simulink model "LabC_CompensatorOverRobot"  (R2017a)
settings: Solver=FixedStepDiscrete  StartTime=0.0  StopTime=inf  FixedStep=fSamplingPeriod  RelTol=1e-3  EnableMultiTasking=on
values from neighbouring files (symbols this model uses):
  Ad = [ ... (first row only)    [LabB_ObserverOverSimulator_Discrete_Parameters.m]
  Bd = [0,           0 ... (first row only)    [LabA_equations.m]    (also in LabB_ObserverOverSimulator_Discrete_Parameters.m = [)
  Cd = [ ... (first row only)    [LabB_ObserverOverSimulator_Discrete_Parameters.m]
  fGyroBias = 125.292978208    [GyroBias.mat]    (also in LabB_TuneTheGyro_SaveParameters.m = mean(afGyroBias.signals.values))
  fGyroConversionFactor = -1/131    (= -0.00763358778626)    [LabB_PIDOverRobot_Parameters.m]    (also in LoadRobotParameters.m = 0.00762939453125)
  fSamplingPeriod = 0.01    [LabB_CheckCommunications_Parameters.m]    (also in LabB_ControllerOverSimulator_Discrete_Parameters.m = 0.005; LabB_ObserverOverSimulator_Discrete_Parameters.m = 0.005; LabB_PIDOverRobot_Parameters.m = 0.005; LabB_TuneTheGyro_SaveParameters.m)
  fWheelRadius = 0.0216    [LabB_PIDOverRobot_Parameters.m]    (also in LoadRobotParameters.m)
  iNumberOfEncoderSteps = 720    [LabB_PIDOverRobot_Parameters.m]    (also in LoadRobotParameters.m)
  Kd = [-8.1792  -49.1223  -71.4928  -11.5909]    [LabB_ControllerOverSimulator_Discrete_Parameters.m]
  Ld = [ ... (first row only)    [LabB_ObserverOverSimulator_Discrete_Parameters.m]
  Md1 = [ ... (first row only)    [LabB_ObserverOverSimulator_Discrete_Parameters.m]
  Md2 = [ ... (first row only)    [LabB_ObserverOverSimulator_Discrete_Parameters.m]
  Md3 = 1.0e+03 * [ ... (first row only)    [LabB_ObserverOverSimulator_Discrete_Parameters.m]
  Md4 = [ ... (first row only)    [LabB_ObserverOverSimulator_Discrete_Parameters.m]
  Md5 = 1.0e+03 * [ ... (first row only)    [LabB_ObserverOverSimulator_Discrete_Parameters.m]
  Md6 = [ ... (first row only)    [LabB_ObserverOverSimulator_Discrete_Parameters.m]
  Md7 = [ ... (first row only)    [LabB_ObserverOverSimulator_Discrete_Parameters.m]
undefined symbols (not defined in the file or in its folder): DiscIntNeverNeededParam, Nud, Nxd, sigbuilder_block
libraries: simulink x16, cstblocks x2, MinSegLibrary_M2V3 x2, arduinolib x1
settings Model: FPTRunName=FPA_Reference  SimulationMode=external  ExtModeTrigDuration=2  Creator=Alec  LastModifiedBy=damiano
settings DataIOCC: SaveFormat=Array  SaveOutput=off  SignalLogging=off  DSMLogging=off  SaveTime=off
settings OptimizationCC: PassReuseOutputArgsAs=Individual arguments  ExpressionDepthLimit=2147483647  MaxStackSize=64
settings DebuggingCC: UnderspecifiedInitializationDetection=Classic  MergeDetectMultiDrivingBlocksExec=none  ParameterTunabilityLossMsg=error  StateNameClashWarn=warning  SFUnexpectedBacktrackingDiag=warning  SFNoUnconditionalDefaultTransitionDiag=warning  SFExecutionAtInitializationDiag=none
settings HardwareCC: ProdBitPerInt=16  ProdBitPerPointer=16  ProdBitPerSizeT=16  ProdBitPerPtrDiffT=16  ProdLargestAtomicFloat=None  ProdWordSize=8  ProdHWDeviceType=Atmel->AVR
settings ModelReferenceCC: PropagateSignalLabelsOutOfModel=off
settings SFSimCC: MATLABDynamicMemAlloc=off
settings RTWCC: SystemTargetFile=ert.tlc  HardwareBoard=Arduino Mega 2560  TLCOptions=-aInlineSetEventsForThisBaseRateFcn=TLC_FALSE -aSuppressMultiTaskScheduler=TLC_FALSE -aRateBasedStepFcn=1  TemplateMakefile=ert_default_tmf  Description=Embedded Coder  GenerateReport=on  RTWVerbose=off  Toolchain=Arduino AVR  BuildConfiguration=Faster Runs  IncludeHyperlinkInReport=on  LaunchReport=on  GenerateTraceInfo=on  GenerateTraceReport=on  GenerateTraceReportSl=on  GenerateTraceReportSf=on  GenerateTraceReportEml=on
settings CodeAppCC: ForceParamTrailComments=on  IgnoreCustomStorageClasses=off  OperatorAnnotations=on  SimulinkDataObjDesc=on  SFDataObjDesc=on  MATLABFcnDesc=on  CustomSymbolStrType=$N$R$M  InsertBlockDesc=on  MATLABSourceComments=on  InternalIdentifier=Classic
settings ERTTargetCC: SupportContinuousTime=on  SupportVariableSizeSignals=on
settings ConfigComp: CovMetricSettings=dw  CovHtmlReporting=on  CovSaveCumulativeToWorkspaceVar=on  CovSaveSingleToWorkspaceVar=on  CovExternalEMLEnable=off

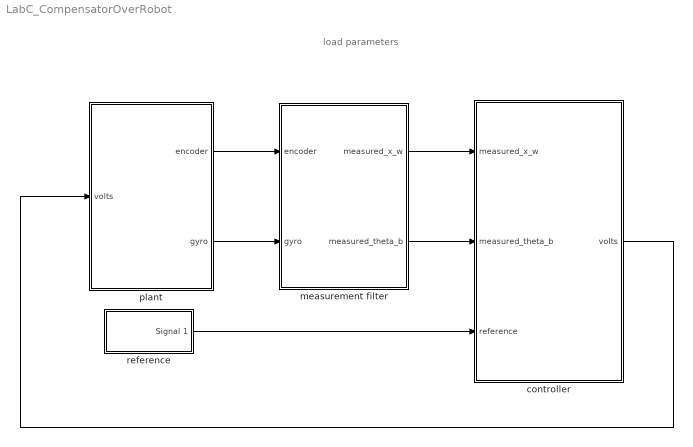
== system LabC_CompensatorOverRobot ==
  note: load parameters
  controller : Subsystem
  measurement filter : Subsystem
  plant : Subsystem
  reference : Subsystem  Tag=STV Subsys  LoadFcn=sigbuilder_block('load');  StartFcn=sigbuilder_block('start');  StopFcn=sigbuilder_block('stop');  ClipboardFcn=sigbuilder_block('clipboard');  mask(Sigbuilder block){tuvar=[0:10]}
      mask help: Simulink:masks:SigbuilderBlock_MD
      mask init:
      | if ~strcmp(get_param(bdroot(gcbh),'SimulationStatus'),'stopped') tuvar = sigbuilder_block('maskInit'); end
      settings: CopyFcn=sigbuilder_block('copy');  DeleteFcn=sigbuilder_block('delete');  ModelCloseFcn=sigbuilder_block('modelClose');  PreSaveFcn=sigbuilder_block('preSave');  PauseFcn=sigbuilder_block('pause');  ContinueFcn=sigbuilder_block('continue');  NameChangeFcn=sigbuilder_block('namechange');  OpenFcn=sigbuilder_block('open',[437.6 199.2 550.4 400 ]);  CloseFcn=sigbuilder_block('close');
      mask Display: plot(0, 0, 100, 100,[2, 2, 32, 32, 2], [68, 8, 8, 68, 68],[32, 2], [38, 38], [32, 19, 2],[53, 60, 44], [32, 17, 17, 2],[16, 16, 31, 31]);txt = getActiveGroup(gcbh);text(2, 100, txt,'verticalAlignment', 'top');
  wires:
  controller/1(volts) -> plant/1(volts)
  measurement filter/2(measured_theta_b) -> controller/2("measured_theta_b ")
  plant/2(gyro) -> measurement filter/2(gyro)
  measurement filter/1(measured_x_w) -> controller/1(measured_x_w)
  plant/1(encoder) -> measurement filter/1(encoder)
  reference/1(Signal 1) -> controller/3(reference)

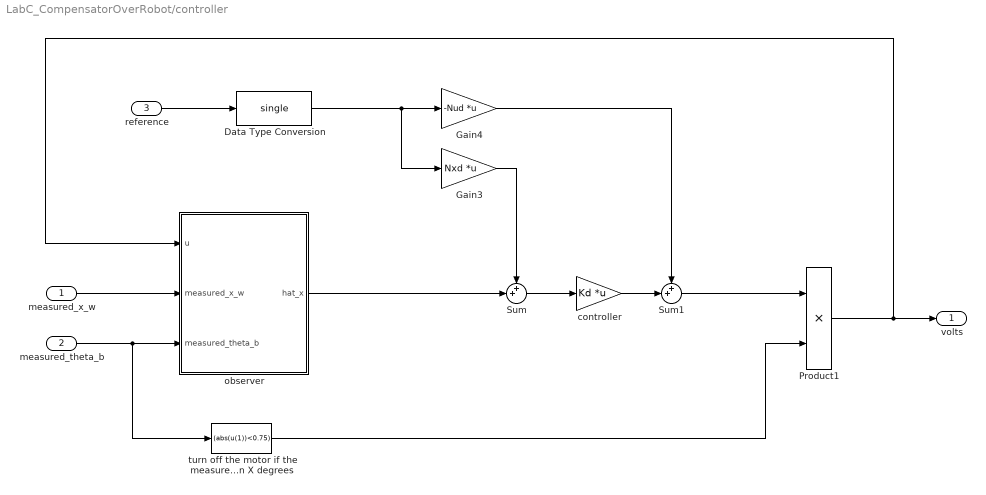
== system LabC_CompensatorOverRobot/controller ==
  measured_x_w : Inport
  "measured_theta_b " : Inport  Port=2
  reference : Inport  Port=3
  Data Type Conversion : DataTypeConversion  OutDataTypeStr=single
  Gain3 : Gain  Gain=Nxd  Multiplication=Matrix(K*u)
  Gain4 : Gain  Gain=-Nud  Multiplication=Matrix(K*u)
  Product1 : Product  RndMeth=Zero
  Sum : Sum  Inputs=++|
  Sum1 : Sum  Inputs=++|
  controller : Gain  Gain=Kd  Multiplication=Matrix(K*u)
  observer : Subsystem
  turn off the motor if the measured angle is greater than X degrees : Fcn  Expr=(abs(u(1))<0.75)
  volts : Outport
  wires:
  turn off the motor if the measured angle is greater than X degrees/1 -> Product1/2
  "measured_theta_b "/1 -> observer/3(measured_theta_b), turn off the motor if the measured angle is greater than X degrees/1
  measured_x_w/1 -> observer/2(measured_x_w)
  Product1/1 -> observer/1(u), volts/1
  Gain3/1 -> Sum/1
  Gain4/1 -> Sum1/1
  reference/1 -> Data Type Conversion/1
  Sum/1 -> controller/1
  controller/1 -> Sum1/2
  Sum1/1 -> Product1/1
  observer/1(hat_x) -> Sum/2
  Data Type Conversion/1 -> Gain3/1, Gain4/1

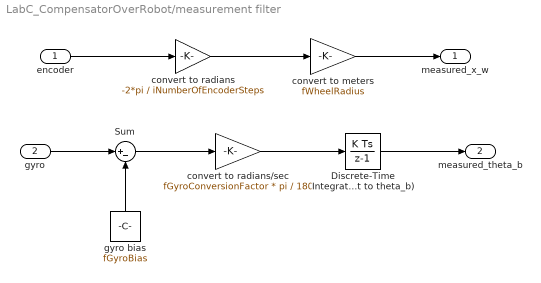
== system LabC_CompensatorOverRobot/measurement filter ==
  encoder : Inport
  gyro : Inport  Port=2
  Discrete-Time Integrator (convert from theta_b_dot to theta_b) : DiscreteIntegrator  SampleTime=fSamplingPeriod  OutDataTypeStr=Inherit: Inherit via back propagation  ICPrevOutput=DiscIntNeverNeededParam  ICPrevScaledInput=DiscIntNeverNeededParam
  Sum : Sum  Inputs=|+-
  convert to radians/sec : Gain  Gain=fGyroConversionFactor * pi / 180  OutDataTypeStr=Inherit: Same as input
  convert to radians : Gain  Gain=-2*pi / iNumberOfEncoderSteps  OutDataTypeStr=Inherit: Same as input
  convert to meters : Gain  Gain=fWheelRadius  OutDataTypeStr=Inherit: Same as input
  gyro bias : Constant  Value=fGyroBias  OutDataTypeStr=single
  measured_x_w : Outport
  measured_theta_b : Outport  Port=2
  wires:
  convert to radians/sec/1 -> Discrete-Time Integrator (convert from theta_b_dot to theta_b)/1
  gyro/1 -> Sum/1
  Sum/1 -> convert to radians/sec/1
  convert to radians/1 -> convert to meters/1
  encoder/1 -> convert to radians/1
  Discrete-Time Integrator (convert from theta_b_dot to theta_b)/1 -> measured_theta_b/1
  gyro bias/1 -> Sum/2
  convert to meters/1 -> measured_x_w/1

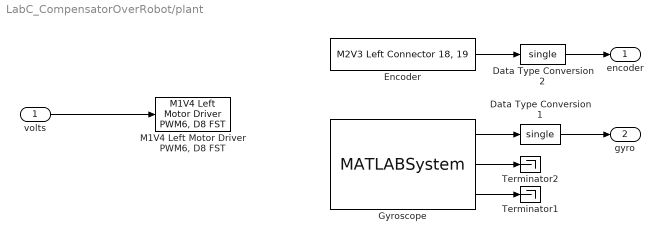
== system LabC_CompensatorOverRobot/plant ==
  volts : Inport
  Data Type Conversion1 : DataTypeConversion  OutDataTypeStr=single
  Data Type Conversion2 : DataTypeConversion  OutDataTypeStr=single
  Encoder : MinSegLibrary_M2V3/M2V3 Left Connector 18, 19  Encoder=1  PinA=19  PinB=18  PWMFSelect=1  PWMTimer=3
      settings: SourceProductName=Rensselaer Arduino Support Package
  Gyroscope : MATLABSystem  System=soMPU6050Gyro  DLPFmode=0
      mask Type: soMPU6050Gyro
      mask Display:
      | disp('soMPU6050Gyro');
      | port_label('output',1,'xvel');
      | port_label('output',2,'yvel');
      | port_label('output',3,'zvel');
  "M1V4 Left Motor Driver PWM6, D8 FST" : MinSegLibrary_M2V3/M1V4 Left Motor Driver PWM6, D8 FST  Vsupply=9
      settings: SourceProductName=Rensselaer Arduino Support Package
  Terminator1 : Terminator
  Terminator2 : Terminator
  encoder : Outport
  gyro : Outport  Port=2
  wires:
  Gyroscope/1 -> Data Type Conversion1/1
  Data Type Conversion1/1 -> gyro/1
  Encoder/1 -> Data Type Conversion2/1
  Data Type Conversion2/1 -> encoder/1
  Gyroscope/3 -> Terminator1/1
  Gyroscope/2 -> Terminator2/1
  volts/1 -> "M1V4 Left Motor Driver PWM6, D8 FST"/1

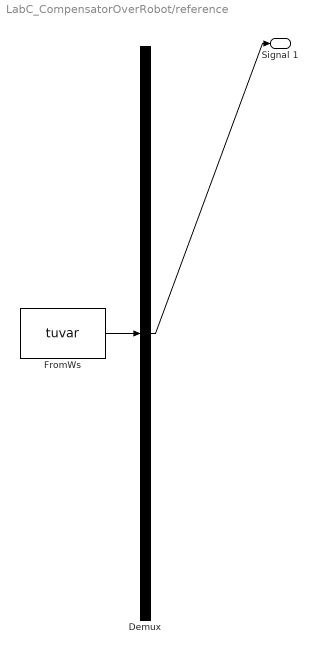
== system LabC_CompensatorOverRobot/reference ==
  Demux : Demux  Tag=STV Demux  Outputs=1
  FromWs : FromWorkspace  Tag=STV FromWs  VariableName=tuvar  SampleTime=0
      SigBuilderData=|
      | common.afterFinalStr = 'Extrapolate'
      | common.sampleTime = 0
      | dataSet.timeRange = [0 120]
      | dataSet.name = 'Group 1'
      | sbobj.Groups.Name = 'Group 1'
      | sbobj.Groups.Signals.Name = 'Signal 1'
      | sbobj.Groups.Signals.XData = [0 10 60 120]
      | sbobj.Groups.Signals.YData = [0 0 2.5 0]
      | sbobj.Groups.TimeRange = [0 120]
  Signal 1 : Outport  Tag=STV Outport
  wires:
  FromWs/1 -> Demux/1
  Demux/1 -> Signal 1/1

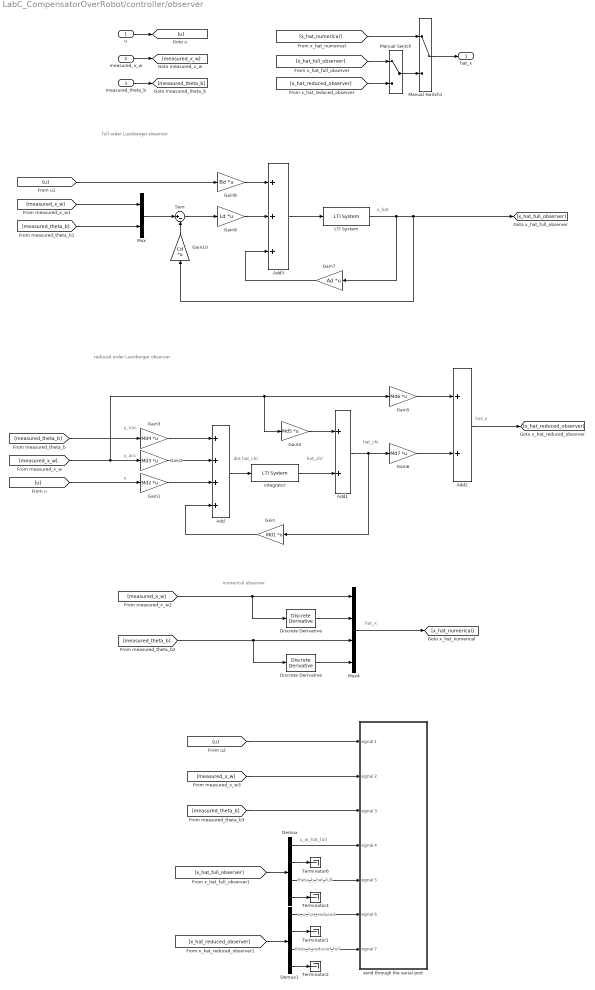
== system LabC_CompensatorOverRobot/controller/observer ==
  note: x_w_hat_full
  note: full order Luenberger observer
  note: reduced order Luenberger observer
  note: numerical observer
  note: hat_x
  note: hat_chi
  note: u
  note: dot hat_chi'
  note: hat_chi'
  note: y_acc
  note: y_nac
  note: x_hat
  note: hat_x
  note: x_w_hat_reduced
  note: theta_b_hat_full
  note: theta_b_reduced_full
  u : Inport
  measured_x_w : Inport  Port=2
  measured_theta_b : Inport  Port=3
  Add : Sum  Inputs=++++
  Add1 : Sum
  Add2 : Sum
  Add3 : Sum  Inputs=+++
  Demux : Demux
  Demux1 : Demux
  Discrete Derivative : simulink/Discrete/Discrete Derivative  gainval=1.0  ICPrevScaledInput=0.0  InputProcessing=Inherited  OutMin=[]  OutMax=[]  OutDataType=fixdt(1, 16)  OutScaling=2^-10  DoSatur=off
  "Discrete Derivative " : simulink/Discrete/Discrete Derivative  gainval=1.0  ICPrevScaledInput=0.0  InputProcessing=Inherited  OutMin=[]  OutMax=[]  OutDataType=fixdt(1, 16)  OutScaling=2^-10  DoSatur=off
  Gain : Gain  Gain=Md1  Multiplication=Matrix(K*u)
  Gain1 : Gain  Gain=Md2  Multiplication=Matrix(K*u)
  Gain10 : Gain  Gain=Cd  Multiplication=Matrix(K*u)
  Gain2 : Gain  Gain=Md3  Multiplication=Matrix(K*u)
  Gain3 : Gain  Gain=Md4  Multiplication=Matrix(K*u)
  Gain4 : Gain  Gain=Md5  Multiplication=Matrix(K*u)
  Gain5 : Gain  Gain=Md6  Multiplication=Matrix(K*u)
  Gain6 : Gain  Gain=Md7  Multiplication=Matrix(K*u)
  Gain7 : Gain  Gain=Ad  Multiplication=Matrix(K*u)
  Gain8 : Gain  Gain=Bd  Multiplication=Matrix(K*u)
  Gain9 : Gain  Gain=Ld  Multiplication=Matrix(K*u)
  LTI System : cstblocks/LTI System  sys=tf(1,[1 0],fSamplingPeriod)*eye(size(Ad))  IC=[]
  Manual Switch : ManualSwitch
  Manual Switch1 : ManualSwitch
  Mux : Mux  Inputs=2
  Mux4 : Mux
  Sum : Sum  Inputs=|+-
  Terminator{1..2,4,6} (4 alike) : Terminator
  integrator : cstblocks/LTI System  sys=tf(1,[1 0],fSamplingPeriod)*eye(3)  IC=[]
  send through the serial port : Subsystem
  hat_x : Outport
  wires:
  Gain3/1 -> Add/1
  Gain2/1 -> Add/2
  Add/1 -> integrator/1
  Gain4/1 -> Add1/1
  Gain1/1 -> Add/3
  Gain/1 -> Add/4
  integrator/1 -> Add1/2
  Add1/1 -> Gain/1, Gain6/1
  Gain5/1 -> Add2/1
  Gain6/1 -> Add2/2
  Discrete Derivative/1 -> Mux4/2
  "Discrete Derivative "/1 -> Mux4/4
  [measured_x_w] -> Gain4/1, Gain5/1, Gain2/1
  [measured_theta_b] -> Gain3/1
  Gain9/1 -> Add3/2
  Sum/1 -> Gain9/1
  [u] -> Gain1/1
  Gain8/1 -> Add3/1
  Gain10/1 -> Sum/2
  Mux/1 -> Sum/1
  Gain7/1 -> Add3/3
  LTI System/1 -> [x_hat_full_observer], Gain10/1, Gain7/1
  Add3/1 -> LTI System/1
  u/1 -> [u]
  measured_x_w/1 -> [measured_x_w]
  measured_theta_b/1 -> [measured_theta_b]
  [u] -> Gain8/1
  [measured_x_w] -> Mux/1
  [measured_theta_b] -> Mux/2
  [measured_x_w] -> Discrete Derivative/1, Mux4/1
  [measured_theta_b] -> "Discrete Derivative "/1, Mux4/3
  [u] -> send through the serial port/1(signal 1)
  [measured_x_w] -> send through the serial port/2(signal 2)
  [measured_theta_b] -> send through the serial port/3(signal 3)
  Mux4/1 -> [x_hat_numerical]
  [x_hat_full_observer] -> Manual Switch/1
  Manual Switch/1 -> Manual Switch1/2
  Manual Switch1/1 -> hat_x/1
  Add2/1 -> [x_hat_reduced_observer]
  [x_hat_reduced_observer] -> Manual Switch/2
  [x_hat_numerical] -> Manual Switch1/1
  [x_hat_full_observer] -> Demux/1
  Demux/1 -> send through the serial port/4(signal 4)
  Demux/3 -> send through the serial port/5(signal 5)
  Demux1/3 -> send through the serial port/7(signal 7)
  Demux1/1 -> send through the serial port/6(signal 6)
  [x_hat_reduced_observer] -> Demux1/1
  Demux/2 -> Terminator6/1
  Demux/4 -> Terminator4/1
  Demux1/2 -> Terminator1/1
  Demux1/4 -> Terminator2/1

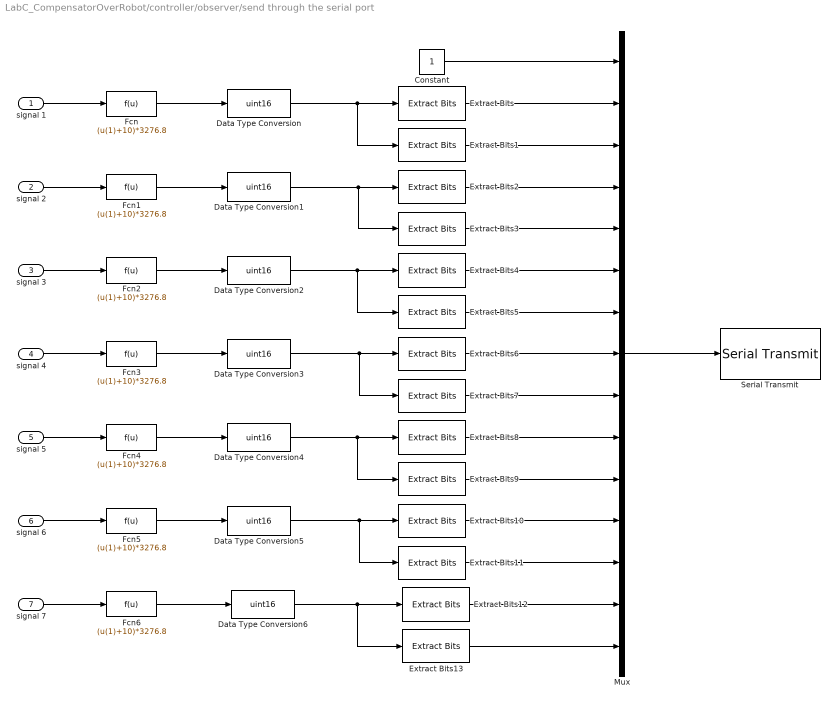
== system LabC_CompensatorOverRobot/controller/observer/send through the serial port ==
  signal 1 : Inport
  signal 2 : Inport  Port=2
  signal 3 : Inport  Port=3
  signal 4 : Inport  Port=4
  signal 5 : Inport  Port=5
  signal 6 : Inport  Port=6
  signal 7 : Inport  Port=7
  Constant : Constant  OutDataTypeStr=uint8
  Data Type Conversion{,1..6} (7 alike) : DataTypeConversion  OutDataTypeStr=uint16
  Extract Bits{,2,4,6,8,10,12} (7 alike) : simulink/Logic and Bit Operations/Extract Bits  bitsToExtract=Upper half  numBits=8  bitIdxRange=[0 7]  outScalingMode=Treat bit field as an integer
      settings: SourceProductName=Simulink
  Extract Bits{1,3,5,7,9,11,13} (7 alike) : simulink/Logic and Bit Operations/Extract Bits  bitsToExtract=Lower half  numBits=8  bitIdxRange=[0 7]  outScalingMode=Treat bit field as an integer
      settings: SourceProductName=Simulink
  Fcn{,1..6} (7 alike) : Fcn  Expr=(u(1)+10)*3276.8
  Mux : Mux  Inputs=15
  Serial Transmit : arduinolib/Serial Transmit  portNumber=0  sendmode=write  sendformat=Decimal  floatprecision=2  blockPlatform=arduino
      settings: SourceProductName=Simulink Support Package for Arduino Hardware
  wires:
  Data Type Conversion/1 -> Extract Bits1/1, Extract Bits/1
  Extract Bits/1 -> Mux/2
  Fcn1/1 -> Data Type Conversion1/1
  Fcn/1 -> Data Type Conversion/1
  Extract Bits2/1 -> Mux/4
  Constant/1 -> Mux/1
  Data Type Conversion1/1 -> Extract Bits2/1, Extract Bits3/1
  Extract Bits1/1 -> Mux/3
  Mux/1 -> Serial Transmit/1
  Extract Bits3/1 -> Mux/5
  Data Type Conversion3/1 -> Extract Bits6/1, Extract Bits7/1
  Extract Bits4/1 -> Mux/6
  Data Type Conversion2/1 -> Extract Bits5/1, Extract Bits4/1
  Extract Bits5/1 -> Mux/7
  Extract Bits6/1 -> Mux/8
  Fcn3/1 -> Data Type Conversion3/1
  Extract Bits7/1 -> Mux/9
  Fcn2/1 -> Data Type Conversion2/1
  Data Type Conversion4/1 -> Extract Bits9/1, Extract Bits8/1
  Fcn5/1 -> Data Type Conversion5/1
  Extract Bits8/1 -> Mux/10
  Extract Bits9/1 -> Mux/11
  Data Type Conversion5/1 -> Extract Bits10/1, Extract Bits11/1
  Extract Bits11/1 -> Mux/13
  Extract Bits10/1 -> Mux/12
  Fcn4/1 -> Data Type Conversion4/1
  signal 2/1 -> Fcn1/1
  signal 7/1 -> Fcn6/1
  signal 6/1 -> Fcn5/1
  signal 3/1 -> Fcn2/1
  signal 1/1 -> Fcn/1
  signal 4/1 -> Fcn3/1
  signal 5/1 -> Fcn4/1
  Extract Bits13/1 -> Mux/15
  Extract Bits12/1 -> Mux/14
  Fcn6/1 -> Data Type Conversion6/1
  Data Type Conversion6/1 -> Extract Bits12/1, Extract Bits13/1
